simulink model "AEB_NEW"  (R2024b)
settings: Solver=VariableStepAuto  StartTime=0.0  StopTime=6  RelTol=1e-3
libraries: simulink x5
settings Model: Creator=Hossam  LastModifiedBy=Hossam
settings SolverCC: ZeroCrossAlgorithm=Adaptive
settings DebuggingCC: IgnoredZcDiagnostic=none

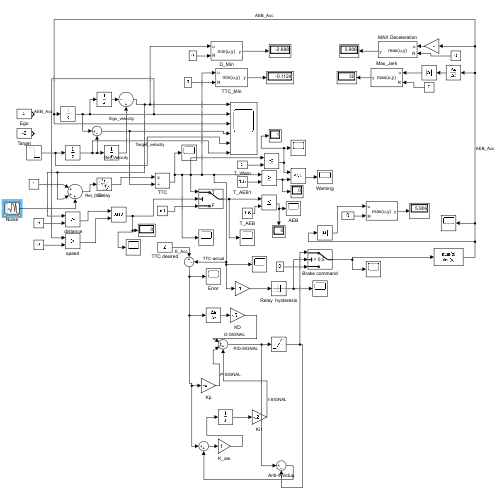
[thumbnail: Simulink's stored preview of the top-level diagram]
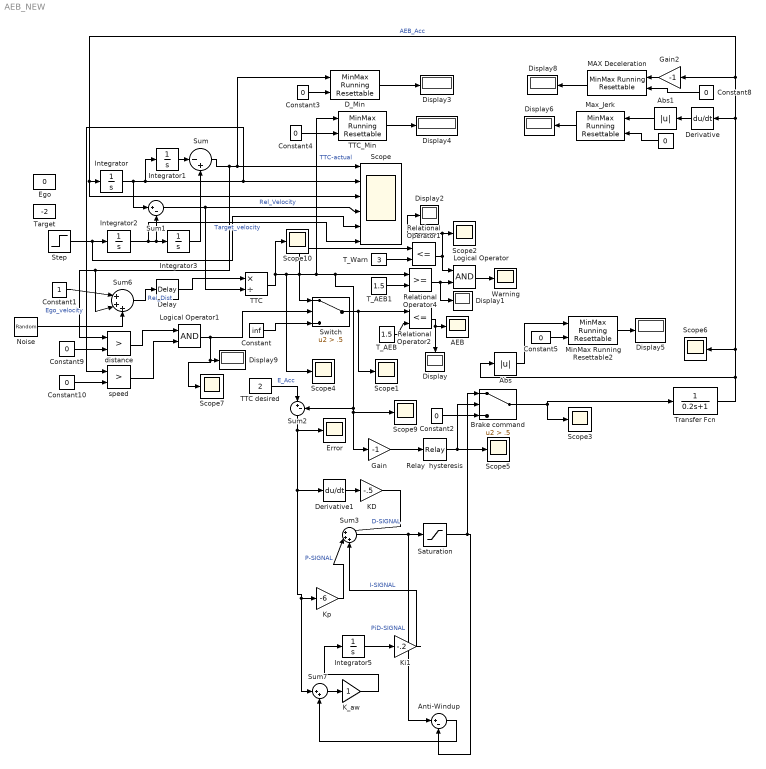
== system AEB_NEW ==
  " MAX Deceleration" : simulink/Math Operations/MinMax Running Resettable  Function=max  vinit=0
  " " : Constant  Value=0
  " distance" : RelationalOperator  Operator=>  OutDataTypeStr=boolean  RndMeth=Simplest  InputSameDT=off
  AEB : Scope
  Abs : Abs  SaturateOnIntegerOverflow=off
  Abs1 : Abs  SaturateOnIntegerOverflow=off
  Anti-Windup : Sum  Inputs=|+-
  Brake command : Switch  Criteria=u2 > Threshold  Threshold=.5  SaturateOnIntegerOverflow=off  InputSameDT=off
  Constant : Constant  Value=inf
  Constant1 : Constant
  Constant{2..5,8..10} (7 alike) : Constant  Value=0
  D_Min : simulink/Math Operations/MinMax Running Resettable  Function=min  vinit=60.0
  Delay : TransportDelay  DelayTime=0.1  InitialOutput=60
  Derivative : Derivative
  Derivative1 : Derivative
  Display{,1..6,8..9} (9 alike) : Display
  Ego : Constant  Value=0
  Error : Scope
  Gain : Gain  Gain=-1
  Gain2 : Gain  Gain=-1
  Integrator : Integrator  InitialCondition=20
  Integrator1 : Integrator
  Integrator2 : Integrator  InitialCondition=10
  Integrator3 : Integrator  InitialCondition=60
  Integrator5 : Integrator
  KD : Gain  Gain=-.5
  K_aw : Gain
  Ki1 : Gain  Gain=-.2
  Kp : Gain  Gain=-6
  Logical Operator : Logic  AllPortsSameDT=off  OutDataTypeStr=boolean
  Logical Operator1 : Logic  AllPortsSameDT=off  OutDataTypeStr=boolean
  Max_Jerk : simulink/Math Operations/MinMax Running Resettable  Function=max  vinit=0
  MinMax Running Resettable2 : simulink/Math Operations/MinMax Running Resettable  Function=max  vinit=0
  Noise : RandomNumber  Variance=.25  Seed=1  SampleTime=0.01
  Relational Operator1 : RelationalOperator  Operator=<=  OutDataTypeStr=boolean  RndMeth=Simplest  InputSameDT=off
  Relational Operator2 : RelationalOperator  Operator=<=  OutDataTypeStr=boolean  RndMeth=Simplest  InputSameDT=off
  Relational Operator4 : RelationalOperator  OutDataTypeStr=boolean  RndMeth=Simplest  InputSameDT=off
  Relay  hysteresis : Relay  OnSwitchValue=-1.5  OffSwitchValue=-2
  Saturation : Saturate  UpperLimit=0  LowerLimit=-6
  Scope : Scope  NumInputPorts=6
  Scope{1..7,9..10} (9 alike) : Scope
  Step : Step  Time=4  After=-2  SampleTime=0
  Sum : Sum  Inputs=|-+
  Sum1 : Sum  Inputs=|+-
  Sum2 : Sum  Inputs=|+-
  Sum3 : Sum  Inputs=|+++
  Sum6 : Sum  Inputs=|+++
  Sum7 : Sum  Inputs=|++
  Switch : Switch  Criteria=u2 > Threshold  Threshold=.5  SaturateOnIntegerOverflow=off  InputSameDT=off
  TTC : Product  Inputs=*/
  TTC desired : Constant  Value=2
  TTC_Min : simulink/Math Operations/MinMax Running Resettable  Function=min  vinit=inf
  T_AEB : Constant  Value=1.5
  T_AEB1 : Constant  Value=1.5
  T_Warn : Constant  Value=3
  Target : Constant  Value=-2
  Transfer Fcn : TransferFcn  Denominator=[0.2 1]
  Warning : Scope
  "speed " : RelationalOperator  Operator=>  OutDataTypeStr=boolean  RndMeth=Simplest  InputSameDT=off
  wires:
  Integrator/1 -> Sum1/1, "speed "/1, Scope/2, Integrator1/1  "Ego_velocity"
  Integrator2/1 -> Scope/6, Sum1/2, Integrator3/1  "Target_velocity"
  Integrator3/1 -> Sum/2
  Sum/1 -> D_Min/1, Scope/1, Sum6/2, " distance"/1
  Sum1/1 -> TTC/2, Scope/4  "Rel_Velocity"
  Integrator1/1 -> Sum/1
  Constant/1 -> Switch/3
  Switch/1 -> Relational Operator2/1, Scope1/1
  T_Warn/1 -> Relational Operator1/2
  Relational Operator1/1 -> Display2/1, Scope2/1, Logical Operator/1
  T_AEB/1 -> Relational Operator2/2
  Relational Operator2/1 -> Display/1, AEB/1
  T_AEB1/1 -> Relational Operator4/2
  Relational Operator4/1 -> Display1/1, Logical Operator/2
  Logical Operator/1 -> Warning/1
  Constant2/1 -> Brake command/3
  Brake command/1 -> Transfer Fcn/1, Scope3/1
  D_Min/1 -> Display3/1
  Constant3/1 -> D_Min/2
  Constant4/1 -> TTC_Min/2
  TTC_Min/1 -> Display4/1
  Constant5/1 -> MinMax Running Resettable2/2
  Abs/1 -> MinMax Running Resettable2/1
  MinMax Running Resettable2/1 -> Display5/1
  Max_Jerk/1 -> Display6/1
  Transfer Fcn/1 -> Gain2/1, Integrator/1, Scope/3, Derivative/1, Scope6/1, Abs/1  "AEB_Acc"
  Gain/1 -> Relay  hysteresis/1
  Derivative/1 -> Abs1/1
  Relay  hysteresis/1 -> Scope5/1, Brake command/2
  TTC/1 -> Scope10/1, Relational Operator4/1, Gain/1, Scope9/1, Sum2/2, TTC_Min/1, Switch/1, Relational Operator1/1, Scope4/1  "TTC-actual"
  TTC desired/1 -> Sum2/1  "E_Acc"
  Sum2/1 -> Error/1, Kp/1, Sum7/1, Derivative1/1
  Constant8/1 -> " MAX Deceleration"/2
  " MAX Deceleration"/1 -> Display8/1
  Gain2/1 -> " MAX Deceleration"/1
  Constant9/1 -> " distance"/2
  Constant10/1 -> "speed "/2
  " distance"/1 -> Logical Operator1/1
  "speed "/1 -> Logical Operator1/2
  Logical Operator1/1 -> Switch/2, Scope7/1, Display9/1
  Step/1 -> Scope/5, Integrator2/1
  " "/1 -> Max_Jerk/2
  Abs1/1 -> Max_Jerk/1
  Constant1/1 -> Sum6/1
  Anti-Windup/1 -> Sum7/2
  Kp/1 -> Sum3/2  "P-SIGNAL"
  Saturation/1 -> Brake command/1, Anti-Windup/2
  Sum7/1 -> K_aw/1
  K_aw/1 -> Integrator5/1
  Derivative1/1 -> KD/1
  KD/1 -> Sum3/1  "D-SIGNAL"
  Sum3/1 -> Saturation/1, Anti-Windup/1  "PiD-SIGNAL"
  Integrator5/1 -> Ki1/1
  Ki1/1 -> Sum3/3  "I-SIGNAL"
  Noise/1 -> Sum6/3
  Sum6/1 -> Delay/1  "Rel_Dist"
  Delay/1 -> TTC/1
